simulink model "MMC_Rectifier_NLM_2018"  (R2023b)
settings: Solver=ode23t  StartTime=0.0  StopTime=3  RelTol=1e-3
libraries: spsIGBTDiodeLib x216, spsSeriesRLCBranchLib x117, spsVoltageMeasurementLib x110, spsCurrentMeasurementLib x7, slpidlib x6, spsThreePhaseVIMeasurementLib x2, spsGroundLib x1, spsPower3phInstantaneousLib x1, spsThreePhaseProgrammableVoltageSourceLib x1, spsThreePhaseSeriesRLCBranchLib x1, spspowerguiLib x1
(part 5 of 5)

== matlab function MMC_Rectifier_NLM_2018/均压/MATLAB Function3 ==
  settings: updateMethod=DISCRETE
  data: NP input; PWM_P output; NL input; IP input; IL input; VP input; VL input; Ts input; PWM_L output
function [PWM_P,PWM_L] = fcn(NP,NL,IP,IL,VP,VL,Ts)
persistent pwm_p pwm_l
if isempty(pwm_p)
    pwm_p=zeros(18,1);
    pwm_l=zeros(18,1);
end
%满足条件进入
if(Ts==0)
    a=18;
    P=zeros(2,18);
    L=zeros(2,18);
%输入电容替换
for i=1:a
    P(1,i)=VP(i);
    P(2,i)=i;
    L(1,i)=VL(i);
    L(2,i)=i;
end
%冒泡排序法
for i=1:a-1;
    for j=1:a-i
        if P(1,j)>P(1,j+1)
           t1=P(1,j);
           t2=P(2,j);
           P(1,j)=P(1,j+1);
           P(2,j)=P(2,j+1);
           P(1,j+1)=t1;
           P(2,j+1)=t2;
        end
     if L(1,j)>L(1,j+1)
           t1=L(1,j);
           t2=L(2,j);
           L(1,j)=L(1,j+1);
           L(2,j)=L(2,j+1);
           L(1,j+1)=t1;
           L(2,j+1)=t2;
     end
    end
end
 pwm_p=zeros(18,1);
 pwm_l=zeros(18,1);
 %判断桥臂电流方向，确定电容充放电
 if NP<=0
     pwm_p=zeros(18,1);
 elseif NP<a
     if IP>0
         for i=1:NP
             pwm_p(P(2,i),1)=1;
         end
     else
         for i=a-NP+1:a
             pwm_p(P(2,i),1)=1;
         end
     end
 else
     pwm_p=ones(18,1);
 end
 if NL<=0
     pwm_l=zeros(18,1);
 elseif NL<a
     if IL>0
         for i=1:NL
             pwm_l(L(2,i),1)=1;
         end
     else
         for i=a-NL+1:a
             pwm_l(L(2,i),1)=1;
         end
     end
 else
     pwm_l=ones(18,1);
 end
end
PWM_P=pwm_p;
PWM_L=pwm_l;

== matlab function MMC_Rectifier_NLM_2018/坐标变换与锁相环/MATLAB Function1 ==
  data: alpha input; wt input; d output; beta input; q output
function [d,q] = alphabeta_to_dq(alpha,wt,beta)

d=cos(wt)*alpha+sin(wt)*beta;
q=-sin(wt)*alpha+cos(wt)*beta;

== matlab function MMC_Rectifier_NLM_2018/坐标变换与锁相环/MATLAB Function ==
  data: a input; alpha output; b input; c input; beta output
function [alpha,beta] = abc_to_alphabeta(a,b,c)

alpha=(2/3)*(a-b/2-c/2);
beta=(2/3)*((sqrt(3)/2)*(b-c));

== matlab function MMC_Rectifier_NLM_2018/坐标变换与锁相环/MATLAB Function2 ==
  data: a input; alpha output; b input; c input; beta output
function [alpha,beta] = abc_to_alphabeta(a,b,c)

alpha=(2/3)*(a-b/2-c/2);
beta=(2/3)*(sqrt(3)/2)*(b-c);

== matlab function MMC_Rectifier_NLM_2018/坐标变换与锁相环/MATLAB Function3 ==
  data: alpha input; wt input; d output; beta input; q output
function [d,q] = alphabeta_to_dq(alpha,wt,beta)

d=cos(wt)*alpha+sin(wt)*beta;
q=-sin(wt)*alpha+cos(wt)*beta;

== matlab function MMC_Rectifier_NLM_2018/环流抑制器/MATLAB Function ==
  data: a input; d output; b input; c input; wt input; q output
function [d,q] = abc_to_dq(a,b,c,wt)
d=(2/3)*(a*cos(2*wt)+b*cos(2*wt+2*pi/3)+c*cos(2*wt-2*pi/3));
q=(2/3)*(a*sin(2*wt)+b*sin(2*wt+2*pi/3)+c*sin(2*wt-2*pi/3));

== matlab function MMC_Rectifier_NLM_2018/环流抑制器/MATLAB Function1 ==
  data: d input; a output; wt input; q input; b output; c output
function [a,b,c] = dq_to_abc(d,wt,q)
a=cos(2*wt)*d+sin(2*wt)*q;
b=cos(2*wt+2*pi/3)*d+sin(2*wt+2*pi/3)*q;
c=cos(2*wt-2*pi/3)*d+sin(2*wt-2*pi/3)*q;

== matlab function MMC_Rectifier_NLM_2018/双闭环控制/MATLAB Function1 ==
  data: d input; a output; wt input; q input; b output; c output
function [a,b,c] = dq_to_abc(d,wt,q)
a=cos(wt)*d-sin(wt)*q;
b=cos(wt-2*pi/3)*d-sin(wt-2*pi/3)*q;
c=cos(wt+2*pi/3)*d-sin(wt+2*pi/3)*q;

== matlab function MMC_Rectifier_NLM_2018/均压/MATLAB Function2 ==
  settings: updateMethod=DISCRETE
  data: NP input; PWM_P output; NL input; IP input; IL input; VP input; VL input; Ts input; PWM_L output
function [PWM_P,PWM_L] = fcn(NP,NL,IP,IL,VP,VL,Ts)
persistent pwm_p pwm_l
if isempty(pwm_p)
    pwm_p=zeros(18,1);
    pwm_l=zeros(18,1);
end
%满足条件进入
if(Ts==0)
    a=18;
    P=zeros(2,18);
    L=zeros(2,18);
%输入电容替换
for i=1:a
    P(1,i)=VP(i);
    P(2,i)=i;
    L(1,i)=VL(i);
    L(2,i)=i;
end
%冒泡排序法
for i=1:a-1;
    for j=1:a-i
        if P(1,j)>P(1,j+1)
           t1=P(1,j);
           t2=P(2,j);
           P(1,j)=P(1,j+1);
           P(2,j)=P(2,j+1);
           P(1,j+1)=t1;
           P(2,j+1)=t2;
        end
     if L(1,j)>L(1,j+1)
           t1=L(1,j);
           t2=L(2,j);
           L(1,j)=L(1,j+1);
           L(2,j)=L(2,j+1);
           L(1,j+1)=t1;
           L(2,j+1)=t2;
     end
    end
end
 pwm_p=zeros(18,1);
 pwm_l=zeros(18,1);
 %判断桥臂电流方向，确定电容充放电
 if NP<=0
     pwm_p=zeros(18,1);
 elseif NP<a
     if IP>0
         for i=1:NP
             pwm_p(P(2,i),1)=1;
         end
     else
         for i=a-NP+1:a
             pwm_p(P(2,i),1)=1;
         end
     end
 else
     pwm_p=ones(18,1);
 end
 if NL<=0
     pwm_l=zeros(18,1);
 elseif NL<a
     if IL>0
         for i=1:NL
             pwm_l(L(2,i),1)=1;
         end
     else
         for i=a-NL+1:a
             pwm_l(L(2,i),1)=1;
         end
     end
 else
     pwm_l=ones(18,1);
 end
end
PWM_P=pwm_p;
PWM_L=pwm_l;
